simulink model "motor_simulink2"  (R2025b)
settings: Solver=FixedStepAuto  StartTime=0.0  StopTime=0.5  FixedStep=1e-6  RelTol=1e-3
undefined symbols (not defined in the file or in its folder): dspblkCoreblockFVToolHelper, gcbh
libraries: slpidlib x4, mcbplantlib x1, autolibpmsminterior x1
settings Model: Creator=wanghuixiang  LastModifiedBy=wanghuixiang

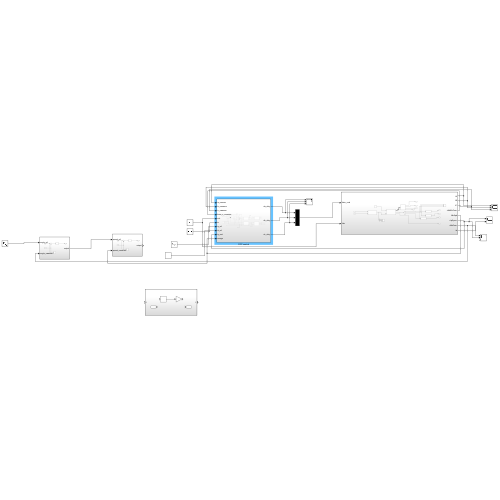
[thumbnail: Simulink's stored preview of the top-level diagram]
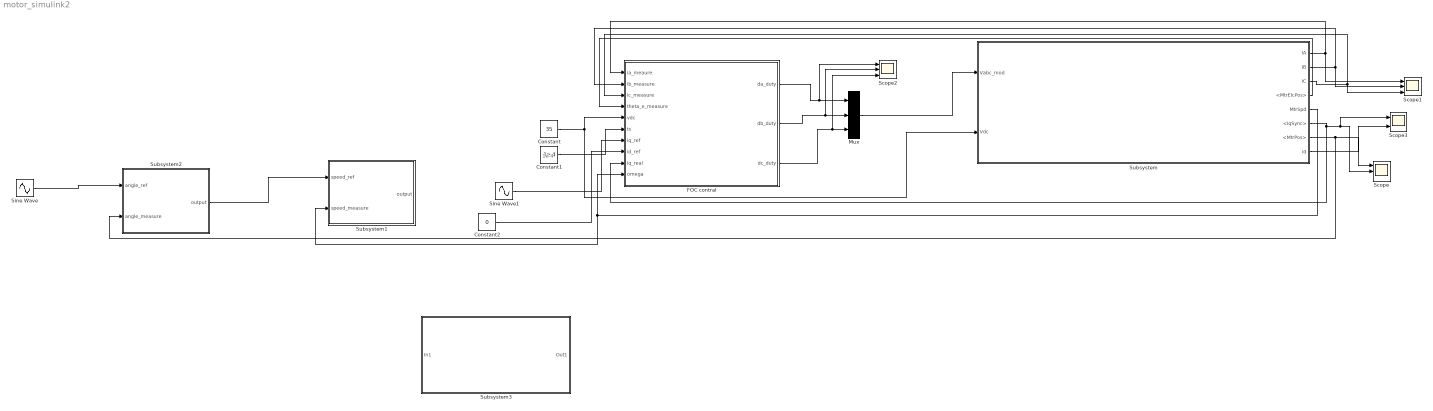
== system motor_simulink2 ==
  note: 1e-4
  Constant : Constant  Value=35
  Constant1 : Constant  Value=1e-4
  Constant2 : Constant  Value=0
  FOC contral : Subsystem
  Mux : Mux  Inputs=3
  Scope : Scope  NumInputPorts=3
      settings: ActiveDisplayYMinimum=-4.2778704038949593  ActiveDisplayYMaximum=5.1731807364811857
  Scope1 : Scope  NumInputPorts=3
      settings: ActiveDisplayYMinimum=-271.31928354066577  ActiveDisplayYMaximum=293.76129527766454
  Scope2 : Scope  NumInputPorts=3
      settings: ActiveDisplayYMinimum=-0.10741833509090637  ActiveDisplayYMaximum=1.0830578553852841  DataLoggingVariableName=ScopeData2
  Scope3 : Scope  NumInputPorts=2
      settings: ActiveDisplayYMinimum=-0.10597587302872147  ActiveDisplayYMaximum=3.0541792317079626  DataLoggingVariableName=ScopeData9
  Sine Wave : Sin  Amplitude=2  Frequency=200  SampleTime=1e-4
  Sine Wave1 : Sin  Amplitude=10  Frequency=300  SampleTime=0
  Subsystem : Subsystem
  Subsystem1 : Subsystem
  Subsystem2 : Subsystem
  Subsystem3 : Subsystem
  wires:
  Constant/1 -> Subsystem/2(Vdc), FOC contral/5(vdc)
  Constant1/1 -> FOC contral/6(ts)
  FOC contral/1(da_duty) -> Mux/1, Scope2/1
  FOC contral/2(db_duty) -> Mux/2, Scope2/2
  FOC contral/3(dc_duty) -> Mux/3, Scope2/3
  Subsystem/1(IA) -> Scope1/1, FOC contral/1(ia_meaure)
  Subsystem/3(IC) -> Scope1/3, FOC contral/3(ic_measure)
  Subsystem/2(IB) -> Scope1/2, FOC contral/2(ib_measure)
  Mux/1 -> Subsystem/1(Vabc_mod)
  Subsystem/6(<IqSync>) -> FOC contral/9(iq_real), Scope3/1, Scope/2
  Subsystem/7(<MtrPos>) -> Subsystem2/2(angle_measure), Scope/1
  Subsystem/8(id) -> Scope3/2
  Subsystem/4(<MtrElcPos>) -> FOC contral/4(theta_e_measure)
  Subsystem/5(MtrSpd) -> FOC contral/10(omega), Subsystem1/2(speed_measure)
  Subsystem2/1(output) -> Subsystem1/1(speed_ref)
  Sine Wave/1 -> Subsystem2/1(angle_ref)
  Constant2/1 -> FOC contral/8(id_ref)
  Sine Wave1/1 -> FOC contral/7(iq_ref)

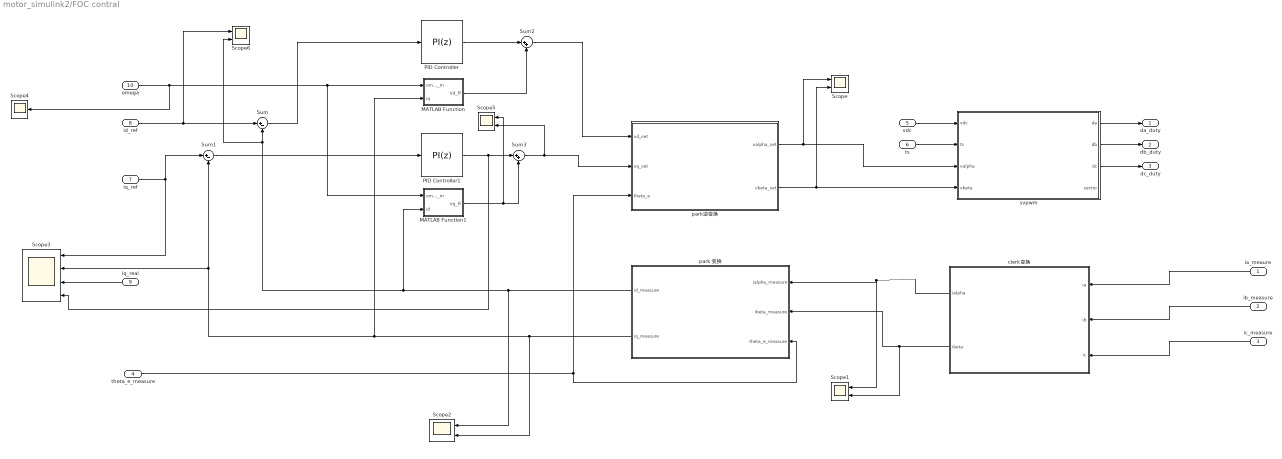
== system motor_simulink2/FOC contral ==
  ia_meaure : Inport
  ib_measure : Inport  Port=2
  ic_measure : Inport  Port=3
  theta_e_measure : Inport  Port=4
  vdc : Inport  Port=5
  ts : Inport  Port=6
  iq_ref : Inport  Port=7
  id_ref : Inport  Port=8
  iq_real : Inport  Port=9
  omega : Inport  Port=10
  MATLAB Function : MATLAB Function  TreatAsAtomicUnit=on
  MATLAB Function1 : MATLAB Function  TreatAsAtomicUnit=on
  PID Controller : slpidlib/PID Controller  Controller=PI  Form=Parallel  TimeDomain=Discrete-time  UseExternalTs=off  SampleTime=1e-4  IntegratorMethod=Forward Euler  FilterMethod=Forward Euler  ControllerParametersSource=internal  P=0.2  I=0  UseKiTs=on  D=0  UseExternalDerivativeSource=off  N=100  UseFilter=on  TunerSelectOption=Transfer Function Based (PID Tuner App)  InitialConditionSource=internal  InitialConditionForIntegrator=0  InitialConditionForFilter=0  DifferentiatorICPrevScaledInput=0  ExternalReset=none  TrackingMode=off  Kt=1  LimitOutput=on  SatLimitsSource=internal  UpperSaturationLimit=19  LowerSaturationLimit=-19  LinearizeAsGain=on  AntiWindupMode=none  Kb=1  LimitIntegrator=on  UpperIntegratorSaturationLimit=19  LowerIntegratorSaturationLimit=-19  POutMin=[]  POutMax=[]  IOutMin=[]  IOutMax=[]  DOutMin=[]  DOutMax=[]  NOutMin=[]  NOutMax=[]  SumOutMin=[]  SumOutMax=[]  SaturationOutMin=[]  SaturationOutMax=[]  PParamMin=[]  PParamMax=[]  IParamMin=[]  IParamMax=[]  DParamMin=[]  DParamMax=[]  NParamMin=[]  NParamMax=[]  KbParamMin=[]  KbParamMax=[]  KtParamMin=[]  KtParamMax=[]  KbOutMin=[]  KbOutMax=[]  KtOutMin=[]  KtOutMax=[]  IntegratorOutMin=[]  IntegratorOutMax=[]  FilterOutMin=[]  FilterOutMax=[]  SumI1OutMin=[]  SumI1OutMax=[]  SumI2OutMin=[]  SumI2OutMax=[]  SumI3OutMin=[]  SumI3OutMax=[]  SumI4OutMin=[]  SumI4OutMax=[]  SumDOutMin=[]  SumDOutMax=[]  DifferentiatorOutMin=[]  DifferentiatorOutMax=[]  FilterDiffOutCoefMin=[]  FilterDiffOutCoefMax=[]  ReciprocalOutMin=[]  ReciprocalOutMax=[]  SumDenOutMin=[]  SumDenOutMax=[]  SumNumOutMin=[]  SumNumOutMax=[]  DivideOutMin=[]  DivideOutMax=[]  UdiffTsProdOutMin=[]  UdiffTsProdOutMax=[]  NTsProdOutMin=[]  NTsProdOutMax=[]  UintegralTsProdOutMin=[]  UintegralTsProdOutMax=[]  UngainTsProdOutMin=[]  UngainTsProdOutMax=[]  ClampingZeroOutDataTypeStr=Inherit: Inherit via back propagation  ClampingZeroOutMin=[]  ClampingZeroOutMax=[]  FilterDenConstantOutDataTypeStr=Inherit: Inherit via back propagation  FilterDenConstantOutMin=[]  FilterDenConstantOutMax=[]  PCopyOutDataTypeStr=Inherit: Inherit via back propagation  PCopyOutMin=[]  PCopyOutMax=[]  NCopyOutDataTypeStr=Inherit: Inherit via back propagation  NCopyOutMin=[]  NCopyOutMax=[]  IntegratorContinuousStateAttributes=''  IntegratorStateMustResolveToSignalObject=off  IntegratorRTWStateStorageClass=Auto  FilterContinuousStateAttributes=''  FilterStateMustResolveToSignalObject=off  FilterRTWStateStorageClass=Auto  ParallelPVariant=InternalParameters  IdealPVariant=Disabled  IVariant=InternalParameters  DVariant=Disabled  IntegratorVariant=Discrete  SatVariant=Enabled  AWVariant=Passthrough  PCopyVariant=Disabled  TRVariant=Disabled  FdbkBlocksVariant=Forward  IdealPFdbkVariant=Disabled  SatFdbkVariant=Disabled  DerivativeFilterVariant=Disabled  NVariant=Disabled  NCopyVariant=Disabled_SignalSpec  FilterICVariant=Disabled  IntegratorICVariant=InternalICs  ExternalResetVariant=Disabled  TRSumVariant=Passthrough  SumFdbkVariant=Disabled  SumVariant=Sum_PI  TsampFilterVariant=InternalTs  TsampNgainVariant=Passthrough  TsampIntegralVariant=Disabled_SignalSpec  ExternalSaturationOutDataTypeStr=Inherit: Same as second input  DerivativeSourceVariant=Disabled  PreIntVariant=InternalPreInt
  PID Controller1 : slpidlib/PID Controller  Controller=PI  Form=Parallel  TimeDomain=Discrete-time  UseExternalTs=off  SampleTime=1e-4  IntegratorMethod=Forward Euler  FilterMethod=Forward Euler  ControllerParametersSource=internal  P=0.2  I=0.002  UseKiTs=on  D=0  UseExternalDerivativeSource=off  N=100  UseFilter=on  TunerSelectOption=Transfer Function Based (PID Tuner App)  InitialConditionSource=internal  InitialConditionForIntegrator=0  InitialConditionForFilter=0  DifferentiatorICPrevScaledInput=0  ExternalReset=none  TrackingMode=off  Kt=1  LimitOutput=on  SatLimitsSource=internal  UpperSaturationLimit=19  LowerSaturationLimit=-19  LinearizeAsGain=on  AntiWindupMode=none  Kb=1  LimitIntegrator=on  UpperIntegratorSaturationLimit=19  LowerIntegratorSaturationLimit=-19  POutMin=[]  POutMax=[]  IOutMin=[]  IOutMax=[]  DOutMin=[]  DOutMax=[]  NOutMin=[]  NOutMax=[]  SumOutMin=[]  SumOutMax=[]  SaturationOutMin=[]  SaturationOutMax=[]  PParamMin=[]  PParamMax=[]  IParamMin=[]  IParamMax=[]  DParamMin=[]  DParamMax=[]  NParamMin=[]  NParamMax=[]  KbParamMin=[]  KbParamMax=[]  KtParamMin=[]  KtParamMax=[]  KbOutMin=[]  KbOutMax=[]  KtOutMin=[]  KtOutMax=[]  IntegratorOutMin=[]  IntegratorOutMax=[]  FilterOutMin=[]  FilterOutMax=[]  SumI1OutMin=[]  SumI1OutMax=[]  SumI2OutMin=[]  SumI2OutMax=[]  SumI3OutMin=[]  SumI3OutMax=[]  SumI4OutMin=[]  SumI4OutMax=[]  SumDOutMin=[]  SumDOutMax=[]  DifferentiatorOutMin=[]  DifferentiatorOutMax=[]  FilterDiffOutCoefMin=[]  FilterDiffOutCoefMax=[]  ReciprocalOutMin=[]  ReciprocalOutMax=[]  SumDenOutMin=[]  SumDenOutMax=[]  SumNumOutMin=[]  SumNumOutMax=[]  DivideOutMin=[]  DivideOutMax=[]  UdiffTsProdOutMin=[]  UdiffTsProdOutMax=[]  NTsProdOutMin=[]  NTsProdOutMax=[]  UintegralTsProdOutMin=[]  UintegralTsProdOutMax=[]  UngainTsProdOutMin=[]  UngainTsProdOutMax=[]  ClampingZeroOutDataTypeStr=Inherit: Inherit via back propagation  ClampingZeroOutMin=[]  ClampingZeroOutMax=[]  FilterDenConstantOutDataTypeStr=Inherit: Inherit via back propagation  FilterDenConstantOutMin=[]  FilterDenConstantOutMax=[]  PCopyOutDataTypeStr=Inherit: Inherit via back propagation  PCopyOutMin=[]  PCopyOutMax=[]  NCopyOutDataTypeStr=Inherit: Inherit via back propagation  NCopyOutMin=[]  NCopyOutMax=[]  IntegratorContinuousStateAttributes=''  IntegratorStateMustResolveToSignalObject=off  IntegratorRTWStateStorageClass=Auto  FilterContinuousStateAttributes=''  FilterStateMustResolveToSignalObject=off  FilterRTWStateStorageClass=Auto  ParallelPVariant=InternalParameters  IdealPVariant=Disabled  IVariant=InternalParameters  DVariant=Disabled  IntegratorVariant=Discrete  SatVariant=Enabled  AWVariant=Passthrough  PCopyVariant=Disabled  TRVariant=Disabled  FdbkBlocksVariant=Forward  IdealPFdbkVariant=Disabled  SatFdbkVariant=Disabled  DerivativeFilterVariant=Disabled  NVariant=Disabled  NCopyVariant=Disabled_SignalSpec  FilterICVariant=Disabled  IntegratorICVariant=InternalICs  ExternalResetVariant=Disabled  TRSumVariant=Passthrough  SumFdbkVariant=Disabled  SumVariant=Sum_PI  TsampFilterVariant=InternalTs  TsampNgainVariant=Passthrough  TsampIntegralVariant=Disabled_SignalSpec  ExternalSaturationOutDataTypeStr=Inherit: Same as second input  DerivativeSourceVariant=Disabled  PreIntVariant=InternalPreInt
  Scope{,1..2,5..6} (5 alike) : Scope  NumInputPorts=2
      Scope settings: ActiveDisplayYMinimum=-5.0548458842177206  ActiveDisplayYMaximum=5.2196458808879767  DataLoggingVariableName=ScopeData3
      Scope1 settings: ActiveDisplayYMinimum=-12.827305709885426  ActiveDisplayYMaximum=13.333371142328733  DataLoggingVariableName=ScopeData4
      Scope2 settings: ActiveDisplayYMinimum=-4.941270004755733  ActiveDisplayYMaximum=8.4835943666230271  DataLoggingVariableName=ScopeData5
      Scope5 settings: ActiveDisplayYMinimum=-15.15417131801717  ActiveDisplayYMaximum=6.09591413502894  DataLoggingVariableName=ScopeData11
      Scope6 settings: ActiveDisplayYMinimum=-0.30479806244928748  ActiveDisplayYMaximum=0.39156695355991433  DataLoggingVariableName=ScopeData13
  Scope3 : Scope  NumInputPorts=4
      settings: ActiveDisplayYMinimum=-8.555590148160233  ActiveDisplayYMaximum=14.026669194501673  DataLoggingVariableName=ScopeData8
  Scope4 : Scope
      settings: ActiveDisplayYMinimum=-748.96819186231789  ActiveDisplayYMaximum=578.08033382458018  DataLoggingVariableName=ScopeData10
  Sum : Sum  Inputs=|+-
  Sum1 : Sum  Inputs=|+-
  Sum2 : Sum  Inputs=|++
  Sum3 : Sum  Inputs=|++
  clerk变换 : MATLAB Function  TreatAsAtomicUnit=on
  park 变换 : MATLAB Function  TreatAsAtomicUnit=on
  park逆变换 : MATLAB Function  TreatAsAtomicUnit=on
  svpwm : MATLAB Function  TreatAsAtomicUnit=on
  da_duty : Outport
  db_duty : Outport  Port=2
  dc_duty : Outport  Port=3
  wires:
  clerk变换/1(ialpha) -> Scope1/1, park 变换/1(ialpha_measure)
  clerk变换/2(ibeta) -> Scope1/2, park 变换/2(ibeta_measure)
  park逆变换/1(valpha_set) -> Scope/1, svpwm/3(valpha)
  park逆变换/2(vbeta_set) -> svpwm/4(vbeta), Scope/2
  theta_e_measure/1 -> park 变换/3(theta_e_measure), park逆变换/3(theta_e)
  svpwm/1(da) -> da_duty/1
  svpwm/2(db) -> db_duty/1
  svpwm/3(dc) -> dc_duty/1
  vdc/1 -> svpwm/1(vdc)
  ts/1 -> svpwm/2(ts)
  park 变换/1(id_measure) -> Scope2/1, MATLAB Function1/2(id), Scope6/2, Sum/2
  id_ref/1 -> Scope6/1, Sum/1
  Sum/1 -> PID Controller/1
  iq_ref/1 -> Scope3/1, Sum1/1
  Sum1/1 -> PID Controller1/1
  park 变换/2(iq_measure) -> Scope2/2, MATLAB Function/2(iq), Sum1/2, Scope3/2
  ia_meaure/1 -> clerk变换/1(ia)
  ib_measure/1 -> clerk变换/2(ib)
  ic_measure/1 -> clerk变换/3(ic)
  iq_real/1 -> Scope3/3
  PID Controller/1 -> Sum2/1
  MATLAB Function/1(Vd_ff) -> Sum2/2
  Sum2/1 -> park逆变换/1(vd_set)
  PID Controller1/1 -> Scope3/4, Sum3/1
  MATLAB Function1/1(Vq_ff) -> Scope5/1, Sum3/2
  Sum3/1 -> Scope5/2, park逆变换/2(vq_set)
  omega/1 -> Scope4/1, MATLAB Function/1(omega_m), MATLAB Function1/1(omega_m)

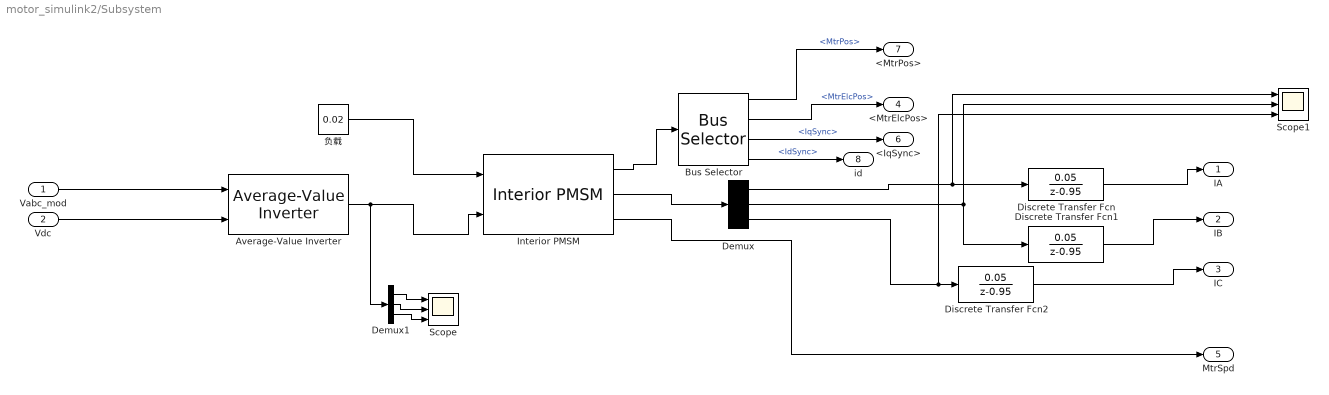
== system motor_simulink2/Subsystem ==
  Vabc_mod : Inport
  Vdc : Inport  Port=2
  Average-Value Inverter : mcbplantlib/Average-Value Inverter
      settings: LibrarySourceBlock=mcblib/Electrical Systems/Inverters/Average-Value Inverter
  Bus Selector : BusSelector  OutputSignals=MtrPos,MtrElcPos,IqSync,IdSync
  Demux : Demux  Outputs=3
  Demux1 : Demux  Outputs=3
  Discrete Transfer Fcn : DiscreteTransferFcn  LoadFcn=dspblkCoreblockFVToolHelper(gcbh,'load');  Numerator=[0.05]  Denominator=[1 -0.95]
      settings: CopyFcn=dspblkCoreblockFVToolHelper(gcbh,'copy');  DeleteFcn=dspblkCoreblockFVToolHelper(gcbh,'close');  ModelCloseFcn=dspblkCoreblockFVToolHelper(gcbh,'close');  PreSaveFcn=dspblkCoreblockFVToolHelper(gcbh,'presave');  PostSaveFcn=dspblkCoreblockFVToolHelper(gcbh,'postsave');  CloseFcn=dspblkCoreblockFVToolHelper(gcbh,'close');
  Discrete Transfer Fcn1 : DiscreteTransferFcn  LoadFcn=dspblkCoreblockFVToolHelper(gcbh,'load');  Numerator=[0.05]  Denominator=[1 -0.95]
      settings: CopyFcn=dspblkCoreblockFVToolHelper(gcbh,'copy');  DeleteFcn=dspblkCoreblockFVToolHelper(gcbh,'close');  ModelCloseFcn=dspblkCoreblockFVToolHelper(gcbh,'close');  PreSaveFcn=dspblkCoreblockFVToolHelper(gcbh,'presave');  PostSaveFcn=dspblkCoreblockFVToolHelper(gcbh,'postsave');  CloseFcn=dspblkCoreblockFVToolHelper(gcbh,'close');
  Discrete Transfer Fcn2 : DiscreteTransferFcn  LoadFcn=dspblkCoreblockFVToolHelper(gcbh,'load');  Numerator=[0.05]  Denominator=[1 -0.95]
      settings: CopyFcn=dspblkCoreblockFVToolHelper(gcbh,'copy');  DeleteFcn=dspblkCoreblockFVToolHelper(gcbh,'close');  ModelCloseFcn=dspblkCoreblockFVToolHelper(gcbh,'close');  PreSaveFcn=dspblkCoreblockFVToolHelper(gcbh,'presave');  PostSaveFcn=dspblkCoreblockFVToolHelper(gcbh,'postsave');  CloseFcn=dspblkCoreblockFVToolHelper(gcbh,'close');
  Interior PMSM : autolibpmsminterior/Interior PMSM  port_config=Torque  sim_type=Discrete  Ts=1e-6  P=7  Rs=0.01709  Ldq=[1e-5, 1.5e-5]  KConstText=Permanent flux linkage constant (lambda_pm):  lambda_pm=0.0036  Ke=159.9771  mechanical=[1e-5, 1e-4, 1e-3]  idq0=[0 0]  theta_init=0  omega_init=0  KConst=0.2205  lambda_pm_calc=0.2205  Kt=0.07  RefBlkName='autolibpmsminterior/Interior PMSM'  aMode=5
      settings: LibrarySourceBlock=mcblib/Electrical Systems/Motors/Interior PMSM
  Scope : Scope  NumInputPorts=3
      settings: ActiveDisplayYMinimum=-22.197081060992033  ActiveDisplayYMaximum=25.053319218494003  DataLoggingVariableName=ScopeData6
  Scope1 : Scope  NumInputPorts=3
      settings: ActiveDisplayYMinimum=-132.21503565487177  ActiveDisplayYMaximum=147.93902485959063  DataLoggingVariableName=ScopeData7
  负载 : Constant  Value=0.02
  IA : Outport
  IB : Outport  Port=2
  IC : Outport  Port=3
  <MtrElcPos> : Outport  Port=4
  MtrSpd : Outport  Port=5
  <IqSync> : Outport  Port=6
  <MtrPos> : Outport  Port=7
  id : Outport  Port=8
  wires:
  Demux/1 -> Scope1/1, Discrete Transfer Fcn/1
  负载/1 -> Interior PMSM/1
  Demux/2 -> Scope1/2, Discrete Transfer Fcn1/1
  Interior PMSM/2 -> Demux/1
  Average-Value Inverter/1 -> Interior PMSM/2, Demux1/1
  Interior PMSM/1 -> Bus Selector/1
  Demux/3 -> Scope1/3, Discrete Transfer Fcn2/1
  Interior PMSM/3 -> MtrSpd/1
  Bus Selector/1 -> <MtrPos>/1  "<MtrPos>"
  Bus Selector/2 -> <MtrElcPos>/1  "<MtrElcPos>"
  Discrete Transfer Fcn/1 -> IA/1
  Discrete Transfer Fcn1/1 -> IB/1
  Discrete Transfer Fcn2/1 -> IC/1
  Demux1/1 -> Scope/1
  Demux1/2 -> Scope/2
  Demux1/3 -> Scope/3
  Vabc_mod/1 -> Average-Value Inverter/1
  Vdc/1 -> Average-Value Inverter/2
  Bus Selector/3 -> <IqSync>/1  "<IqSync>"
  Bus Selector/4 -> id/1  "<IdSync>"

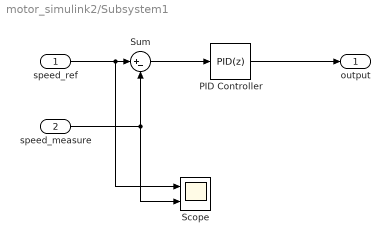
== system motor_simulink2/Subsystem1 ==
  speed_ref : Inport
  speed_measure : Inport  Port=2
  PID Controller : slpidlib/PID Controller  Controller=PID  Form=Parallel  TimeDomain=Discrete-time  UseExternalTs=off  SampleTime=-1  IntegratorMethod=Forward Euler  FilterMethod=Forward Euler  ControllerParametersSource=internal  P=0.2  I=0.0005  UseKiTs=on  D=0.00001  UseExternalDerivativeSource=off  N=100  UseFilter=off  TunerSelectOption=Transfer Function Based (PID Tuner App)  InitialConditionSource=internal  InitialConditionForIntegrator=0  InitialConditionForFilter=0  DifferentiatorICPrevScaledInput=0  ExternalReset=none  TrackingMode=off  Kt=1  LimitOutput=on  SatLimitsSource=internal  UpperSaturationLimit=80  LowerSaturationLimit=-80  LinearizeAsGain=on  AntiWindupMode=none  Kb=1  LimitIntegrator=on  UpperIntegratorSaturationLimit=80  LowerIntegratorSaturationLimit=-80  POutMin=[]  POutMax=[]  IOutMin=[]  IOutMax=[]  DOutMin=[]  DOutMax=[]  NOutMin=[]  NOutMax=[]  SumOutMin=[]  SumOutMax=[]  SaturationOutMin=[]  SaturationOutMax=[]  PParamMin=[]  PParamMax=[]  IParamMin=[]  IParamMax=[]  DParamMin=[]  DParamMax=[]  NParamMin=[]  NParamMax=[]  KbParamMin=[]  KbParamMax=[]  KtParamMin=[]  KtParamMax=[]  KbOutMin=[]  KbOutMax=[]  KtOutMin=[]  KtOutMax=[]  IntegratorOutMin=[]  IntegratorOutMax=[]  FilterOutMin=[]  FilterOutMax=[]  SumI1OutMin=[]  SumI1OutMax=[]  SumI2OutMin=[]  SumI2OutMax=[]  SumI3OutMin=[]  SumI3OutMax=[]  SumI4OutMin=[]  SumI4OutMax=[]  SumDOutMin=[]  SumDOutMax=[]  DifferentiatorOutMin=[]  DifferentiatorOutMax=[]  FilterDiffOutCoefMin=[]  FilterDiffOutCoefMax=[]  ReciprocalOutMin=[]  ReciprocalOutMax=[]  SumDenOutMin=[]  SumDenOutMax=[]  SumNumOutMin=[]  SumNumOutMax=[]  DivideOutMin=[]  DivideOutMax=[]  UdiffTsProdOutMin=[]  UdiffTsProdOutMax=[]  NTsProdOutMin=[]  NTsProdOutMax=[]  UintegralTsProdOutMin=[]  UintegralTsProdOutMax=[]  UngainTsProdOutMin=[]  UngainTsProdOutMax=[]  ClampingZeroOutDataTypeStr=Inherit: Inherit via back propagation  ClampingZeroOutMin=[]  ClampingZeroOutMax=[]  FilterDenConstantOutDataTypeStr=Inherit: Inherit via back propagation  FilterDenConstantOutMin=[]  FilterDenConstantOutMax=[]  PCopyOutDataTypeStr=Inherit: Inherit via back propagation  PCopyOutMin=[]  PCopyOutMax=[]  NCopyOutDataTypeStr=Inherit: Inherit via back propagation  NCopyOutMin=[]  NCopyOutMax=[]  IntegratorContinuousStateAttributes=''  IntegratorStateMustResolveToSignalObject=off  IntegratorRTWStateStorageClass=Auto  FilterContinuousStateAttributes=''  FilterStateMustResolveToSignalObject=off  FilterRTWStateStorageClass=Auto  ParallelPVariant=InternalParameters  IdealPVariant=Disabled  IVariant=InternalParameters  DVariant=InternalParameters  IntegratorVariant=Discrete  SatVariant=Enabled  AWVariant=Passthrough  PCopyVariant=Disabled  TRVariant=Disabled  FdbkBlocksVariant=Forward  IdealPFdbkVariant=Disabled  SatFdbkVariant=Disabled  DerivativeFilterVariant=Differentiator  NVariant=Passthrough  NCopyVariant=Disabled_SignalSpec  FilterICVariant=InternalICsDifferentiator  IntegratorICVariant=InternalICs  ExternalResetVariant=Disabled  TRSumVariant=Passthrough  SumFdbkVariant=Disabled  SumVariant=Sum_PID  TsampFilterVariant=InternalTs  TsampNgainVariant=Passthrough  TsampIntegralVariant=Disabled_SignalSpec  ExternalSaturationOutDataTypeStr=Inherit: Same as second input  DerivativeSourceVariant=ErrorSignal  PreIntVariant=InternalPreInt
  Scope : Scope  NumInputPorts=2
      settings: ActiveDisplayYMinimum=-259.66560264240979  ActiveDisplayYMaximum=336.05516451019355  DataLoggingVariableName=ScopeData12
  Sum : Sum  Inputs=|+-
  output : Outport
  wires:
  speed_measure/1 -> Scope/2, Sum/2
  speed_ref/1 -> Scope/1, Sum/1
  Sum/1 -> PID Controller/1
  PID Controller/1 -> output/1

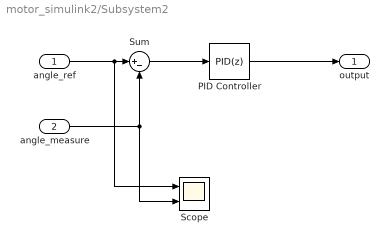
== system motor_simulink2/Subsystem2 ==
  angle_ref : Inport
  angle_measure : Inport  Port=2
  PID Controller : slpidlib/PID Controller  Controller=PID  Form=Parallel  TimeDomain=Discrete-time  UseExternalTs=off  SampleTime=-1  IntegratorMethod=Forward Euler  FilterMethod=Forward Euler  ControllerParametersSource=internal  P=200  I=0.2  UseKiTs=on  D=0  UseExternalDerivativeSource=off  N=100  UseFilter=off  TunerSelectOption=Transfer Function Based (PID Tuner App)  InitialConditionSource=internal  InitialConditionForIntegrator=0  InitialConditionForFilter=0  DifferentiatorICPrevScaledInput=0  ExternalReset=none  TrackingMode=off  Kt=1  LimitOutput=on  SatLimitsSource=internal  UpperSaturationLimit=4000  LowerSaturationLimit=-4000  LinearizeAsGain=on  AntiWindupMode=none  Kb=1  LimitIntegrator=on  UpperIntegratorSaturationLimit=1000  LowerIntegratorSaturationLimit=-1000  POutMin=[]  POutMax=[]  IOutMin=[]  IOutMax=[]  DOutMin=[]  DOutMax=[]  NOutMin=[]  NOutMax=[]  SumOutMin=[]  SumOutMax=[]  SaturationOutMin=[]  SaturationOutMax=[]  PParamMin=[]  PParamMax=[]  IParamMin=[]  IParamMax=[]  DParamMin=[]  DParamMax=[]  NParamMin=[]  NParamMax=[]  KbParamMin=[]  KbParamMax=[]  KtParamMin=[]  KtParamMax=[]  KbOutMin=[]  KbOutMax=[]  KtOutMin=[]  KtOutMax=[]  IntegratorOutMin=[]  IntegratorOutMax=[]  FilterOutMin=[]  FilterOutMax=[]  SumI1OutMin=[]  SumI1OutMax=[]  SumI2OutMin=[]  SumI2OutMax=[]  SumI3OutMin=[]  SumI3OutMax=[]  SumI4OutMin=[]  SumI4OutMax=[]  SumDOutMin=[]  SumDOutMax=[]  DifferentiatorOutMin=[]  DifferentiatorOutMax=[]  FilterDiffOutCoefMin=[]  FilterDiffOutCoefMax=[]  ReciprocalOutMin=[]  ReciprocalOutMax=[]  SumDenOutMin=[]  SumDenOutMax=[]  SumNumOutMin=[]  SumNumOutMax=[]  DivideOutMin=[]  DivideOutMax=[]  UdiffTsProdOutMin=[]  UdiffTsProdOutMax=[]  NTsProdOutMin=[]  NTsProdOutMax=[]  UintegralTsProdOutMin=[]  UintegralTsProdOutMax=[]  UngainTsProdOutMin=[]  UngainTsProdOutMax=[]  ClampingZeroOutDataTypeStr=Inherit: Inherit via back propagation  ClampingZeroOutMin=[]  ClampingZeroOutMax=[]  FilterDenConstantOutDataTypeStr=Inherit: Inherit via back propagation  FilterDenConstantOutMin=[]  FilterDenConstantOutMax=[]  PCopyOutDataTypeStr=Inherit: Inherit via back propagation  PCopyOutMin=[]  PCopyOutMax=[]  NCopyOutDataTypeStr=Inherit: Inherit via back propagation  NCopyOutMin=[]  NCopyOutMax=[]  IntegratorContinuousStateAttributes=''  IntegratorStateMustResolveToSignalObject=off  IntegratorRTWStateStorageClass=Auto  FilterContinuousStateAttributes=''  FilterStateMustResolveToSignalObject=off  FilterRTWStateStorageClass=Auto  ParallelPVariant=InternalParameters  IdealPVariant=Disabled  IVariant=InternalParameters  DVariant=InternalParameters  IntegratorVariant=Discrete  SatVariant=Enabled  AWVariant=Passthrough  PCopyVariant=Disabled  TRVariant=Disabled  FdbkBlocksVariant=Forward  IdealPFdbkVariant=Disabled  SatFdbkVariant=Disabled  DerivativeFilterVariant=Differentiator  NVariant=Passthrough  NCopyVariant=Disabled_SignalSpec  FilterICVariant=InternalICsDifferentiator  IntegratorICVariant=InternalICs  ExternalResetVariant=Disabled  TRSumVariant=Passthrough  SumFdbkVariant=Disabled  SumVariant=Sum_PID  TsampFilterVariant=InternalTs  TsampNgainVariant=Passthrough  TsampIntegralVariant=Disabled_SignalSpec  ExternalSaturationOutDataTypeStr=Inherit: Same as second input  DerivativeSourceVariant=ErrorSignal  PreIntVariant=InternalPreInt
  Scope : Scope  NumInputPorts=2
      settings: ActiveDisplayYMinimum=-16.370748333392054  ActiveDisplayYMaximum=16.327003177893676  DataLoggingVariableName=ScopeData12
  Sum : Sum  Inputs=|+-
  output : Outport
  wires:
  angle_measure/1 -> Scope/2, Sum/2
  angle_ref/1 -> Scope/1, Sum/1
  Sum/1 -> PID Controller/1
  PID Controller/1 -> output/1

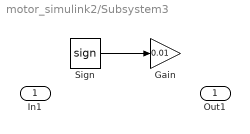
== system motor_simulink2/Subsystem3 ==
  In1 : Inport
  Gain : Gain  Gain=0.01
  Sign : Signum
  Out1 : Outport
  wires:
  Sign/1 -> Gain/1

== matlab function motor_simulink2/FOC contral/park逆变换 ==
  data: vd_set input; valpha_set output; vq_set input; theta_e input; vbeta_set output
function [valpha_set, vbeta_set] = inv_park_transform(vd_set, vq_set, theta_e)
    c = cos(theta_e);
    s = sin(theta_e);
    valpha_set = c*vd_set - s*vq_set;
    vbeta_set  = s*vd_set + c*vq_set;
end

== matlab function motor_simulink2/FOC contral/park 变换 ==
  data: ialpha_measure input; id_measure output; ibeta_measure input; theta_e_measure input; iq_measure output
function [id_measure, iq_measure] = park_transform(ialpha_measure, ibeta_measure, theta_e_measure)
% Park 变换（等幅值）
% 输入：
%   ialpha, ibeta : α-β 轴电流
%   theta_e       : 电角度（rad）
% 输出：
%   id, iq        : d-q 轴电流
    c = cos(theta_e_measure);
    s = sin(theta_e_measure);
    id_measure =  c*ialpha_measure + s*ibeta_measure;
    iq_measure = -s*ialpha_measure + c*ibeta_measure;
end

== matlab function motor_simulink2/FOC contral/clerk变换 ==
  data: ia input; ialpha output; ib input; ibeta output; ic input
function [ialpha, ibeta] = clarke_transform(ia, ib, ic)
% Clarke 正变换（等幅值）
% 输入：ia, ib, ic (三相电流)
% 输出：ialpha, ibeta
% 注意：默认 ia + ib + ic = 0
    
    ialpha = ia;
    ibeta = (1/sqrt(3)) * (ia + 2*ib); 
    % 或者写成：ibeta = (1/sqrt(3)) * (ib - ic);
    % 两者在 ia+ib+ic=0 时完全等价
end

== matlab function motor_simulink2/FOC contral/svpwm ==
  data: vdc input; ts input; valpha input; da output; vbeta input; db output; dc output; sector output
function [da, db, dc, sector] = svpwm( vdc, ts,valpha, vbeta)
%#codegen
% SVPWM（七段式，中心对齐）
% 输入：valpha, vbeta —— 等幅值 Clarke 下的相电压给定
%       vdc           —— 母线电压
%       ts            —— PWM 周期
% 输出：da, db, dc    —— 三相占空比 [0,1]
%       sector        —— 当前扇区（调试用）

    if vdc < 1e-6
        vdc = 1e-6;
    end

    % ---------- 1. 扇区判断 ----------
    vref1 = vbeta;
    vref2 = 0.5*(sqrt(3)*valpha - vbeta);
    vref3 = 0.5*(-sqrt(3)*valpha - vbeta);

    A = vref1 > 0;
    B = vref2 > 0;
    C = vref3 > 0;
    N = A + 2*B + 4*C;

    switch N
        case 3, sector = 1;
        case 1, sector = 2;
        case 5, sector = 3;
        case 4, sector = 4;
        case 6, sector = 5;
        case 2, sector = 6;
        otherwise, sector = 1;   % N=0/7，零矢量附近，兜底
    end

    % ---------- 2. 中间变量 ----------
    X = sqrt(3)*ts*vbeta / vdc;
    Y = ts*(1.5*valpha + 0.5*sqrt(3)*vbeta) / vdc;
    Z = ts*(-1.5*valpha + 0.5*sqrt(3)*vbeta) / vdc;

    % ---------- 3. 作用时间 ----------
    switch sector
        case 1, T1 = -Z; T2 =  X;
        case 2, T1 =  Z; T2 =  Y;
        case 3, T1 =  X; T2 = -Y;
        case 4, T1 = -X; T2 =  Z;
        case 5, T1 = -Y; T2 = -Z;
        case 6, T1 =  Y; T2 = -X;
        otherwise, T1 = 0; T2 = 0;
    end

    % ---------- 4. 过调制限幅 ----------
    if (T1 + T2) > ts
        k  = ts / (T1 + T2);
        T1 = T1 * k;
        T2 = T2 * k;
    end
    if T1 < 0, T1 = 0; end
    if T2 < 0, T2 = 0; end

    % ---------- 5. 切换时间 ----------
    Ta = (ts - T1 - T2) / 4;
    Tb = Ta + T1/2;
    Tc = Tb + T2/2;

    switch sector
        case 1, Tcm1=Ta; Tcm2=Tb; Tcm3=Tc;
        case 2, Tcm1=Tb; Tcm2=Ta; Tcm3=Tc;
        case 3, Tcm1=Tc; Tcm2=Ta; Tcm3=Tb;
        case 4, Tcm1=Tc; Tcm2=Tb; Tcm3=Ta;
        case 5, Tcm1=Tb; Tcm2=Tc; Tcm3=Ta;
        case 6, Tcm1=Ta; Tcm2=Tc; Tcm3=Tb;
        otherwise, Tcm1=Ta; Tcm2=Tb; Tcm3=Tc;
    end

    % ---------- 6. 占空比计算 (已修正) ----------
    % 因为 Tcm 是低电平/零矢量的半周期时间，所以高电平占空比为 1 - 2 * (Tcm/ts)
    da = 1 - 2 * (Tcm1 / ts);
    db = 1 - 2 * (Tcm2 / ts);
    dc = 1 - 2 * (Tcm3 / ts);
end

== matlab function motor_simulink2/FOC contral/MATLAB Function ==
  data: omega_m input; Vd_ff output; iq input
function Vd_ff = d_axis_ff(omega_m, iq)
    % --- 新电机参数 ---
    P = 7;              % 极对数
    Lq = 1.5e-5;        % q轴电感 (H) 已更新
    
    % 计算电角速度
    omega_e = omega_m * P;
    
    % 理论交叉解耦前馈电压
    Vd_ff_raw = -omega_e * Lq * iq;
    
    % --- 防震荡平滑死区 ---
    % 电角速度低于 30 rad/s 完全关闭前馈，30~80 rad/s 线性过渡，80以上全开
    weight = 1;
    % 输出平滑后的前馈电压
    Vd_ff = Vd_ff_raw * weight;
end

== matlab function motor_simulink2/FOC contral/MATLAB Function1 ==
  data: omega_m input; Vq_ff output; id input
function Vq_ff = q_axis_ff(omega_m, id)
    % --- 新电机参数 ---
    P = 7;              % 极对数
    Ld = 1e-5;          % d轴电感 (H) 
    flux = 0.0036;      % 永磁体磁链 (Wb)
    
    % 计算电角速度
    omega_e = omega_m * P;
    
    % 理论前馈电压 (反电动势项 + 交叉解耦项)
    Vq_ff_raw = omega_e * flux + omega_e * Ld * id;
    
    % --- 防震荡平滑死区 (与d轴保持完全同步) ---
    weight = 1;
    % 输出平滑后的前馈电压
    Vq_ff = Vq_ff_raw * weight;
end
